simulink model "Project5_Drivetrain_Edge_Simulink"  (R2022b)
settings: Solver=FixedStepDiscrete  StartTime=0.0  StopTime=14  FixedStep=1.0  RelTol=1e-3
PreLoadFcn:
  | load('Project5_Trained_Workspace.mat');
InitFcn:
  | clear simulinkEdgeInference; load('Project5_Trained_Workspace.mat');
undefined symbols (not defined in the file or in its folder): simulinkEdgeInference
settings Model: Creator=ASUS  LastModifiedBy=ASUS

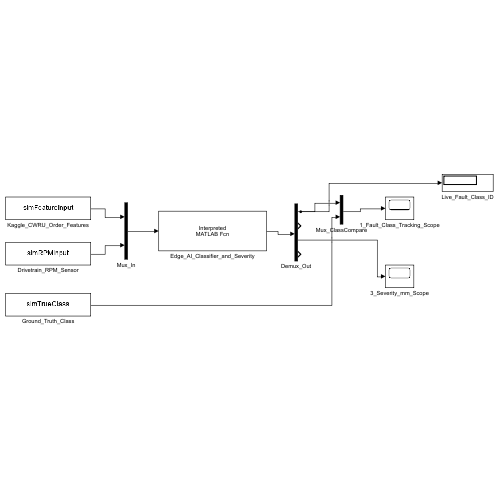
[thumbnail: Simulink's stored preview of the top-level diagram]
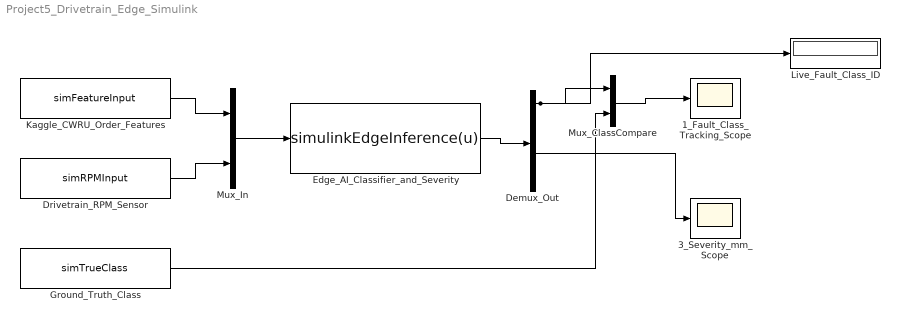
== system Project5_Drivetrain_Edge_Simulink ==
  1_Fault_Class_Tracking_Scope : Scope
  3_Severity_mm_Scope : Scope
  Demux_Out : Demux
  Drivetrain_RPM_Sensor : FromWorkspace  VariableName=simRPMInput  SampleTime=1
  Edge_AI_Classifier_and_Severity : MATLABFcn  MATLABFcn=simulinkEdgeInference(u)  OutputDimensions=4
  Ground_Truth_Class : FromWorkspace  VariableName=simTrueClass  SampleTime=1
  Kaggle_CWRU_Order_Features : FromWorkspace  VariableName=simFeatureInput  SampleTime=1
  Live_Fault_Class_ID : Display
  Mux_ClassCompare : Mux  Inputs=2
  Mux_In : Mux  Inputs=2
  wires:
  Kaggle_CWRU_Order_Features/1 -> Mux_In/1
  Drivetrain_RPM_Sensor/1 -> Mux_In/2
  Mux_In/1 -> Edge_AI_Classifier_and_Severity/1
  Edge_AI_Classifier_and_Severity/1 -> Demux_Out/1
  Demux_Out/1 -> Mux_ClassCompare/1, Live_Fault_Class_ID/1
  Ground_Truth_Class/1 -> Mux_ClassCompare/2
  Mux_ClassCompare/1 -> 1_Fault_Class_Tracking_Scope/1
  Demux_Out/3 -> 3_Severity_mm_Scope/1
